simulink model "Simscape08"  (R2025b)
settings: Solver=ode23t  StartTime=0.0  StopTime=10  RelTol=1e-3
libraries: fl_lib x10, nesl_utility x4
settings Model: Creator=Nico6700  LastModifiedBy=Nico6700

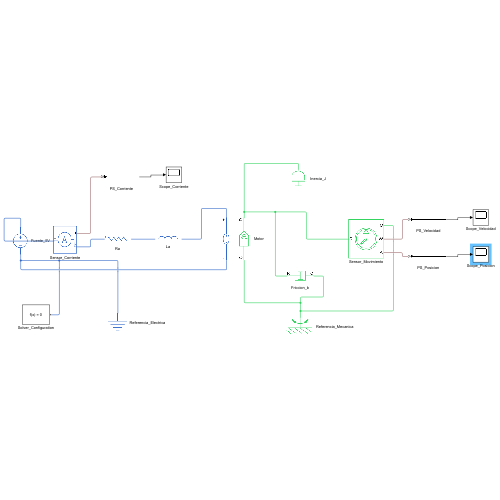
[thumbnail: Simulink's stored preview of the top-level diagram]
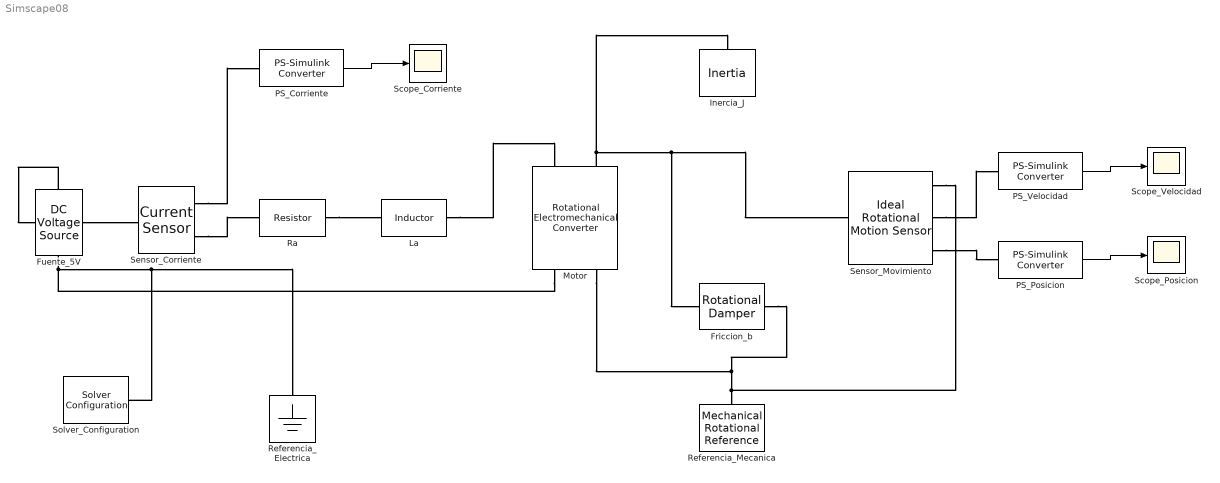
== system Simscape08 ==
  Friccion_b : fl_lib/Mechanical/Rotational Elements/Rotational Damper  D=0.0012 N*m*s/rad  w_specify=off  w_priority=None  w=0 rad/s  w_nominal_specify=off  w_nominal_value=1  w_nominal_unit=rad/s  t_specify=off  t_priority=None  t=0 N*m  t_nominal_specify=off  t_nominal_value=1  t_nominal_unit=N*m
  Fuente_5V : fl_lib/Electrical/Electrical Sources/DC Voltage Source  v0=5 V
  Inercia_J : fl_lib/Mechanical/Rotational Elements/Inertia  inertia=0.001 kg*m^2  num_ports=foundation.enum.numPorts2.one  w_specify=off  w_priority=High  w=0 rad/s  w_nominal_specify=off  w_nominal_value=1  w_nominal_unit=rad/s  t_specify=off  t_priority=None  t=0 N*m  t_nominal_specify=off  t_nominal_value=1  t_nominal_unit=N*m
  La : fl_lib/Electrical/Electrical Elements/Inductor  l=0.023 H  r=0 Ohm  g=1e-9 1/Ohm  i_specify=off  i_priority=None  i=0 A  i_nominal_specify=off  i_nominal_value=1  i_nominal_unit=A  v_specify=off  v_priority=None  v=0 V  v_nominal_specify=off  v_nominal_value=1  v_nominal_unit=V  i_L_specify=off  i_L_priority=High  i_L=0 A  i_L_nominal_specify=off  i_L_nominal_value=1  i_L_nominal_unit=A
  Motor : fl_lib/Electrical/Electrical Elements/Rotational Electromechanical Converter  K=0.01 V*s/rad  i_specify=off  i_priority=None  i=0 A  i_nominal_specify=off  i_nominal_value=1  i_nominal_unit=A  v_specify=off  v_priority=None  v=0 V  v_nominal_specify=off  v_nominal_value=1  v_nominal_unit=V  t_specify=off  t_priority=None  t=0 N*m  t_nominal_specify=off  t_nominal_value=1  t_nominal_unit=N*m  w_specify=off  w_priority=None  w=0 rad/s  w_nominal_specify=off  w_nominal_value=1  w_nominal_unit=rad/s
  PS_Corriente : nesl_utility/PS-Simulink Converter  PhysicalDomain=network_engine_domain  SubClassName=ps_output  LeftPortType=input  RightPortType=output  PseudoPeriodic=off  Frequencies=[]  VectorFormat=inherit  Unit=A  AffineConversion=off
  PS_Posicion : nesl_utility/PS-Simulink Converter  PhysicalDomain=network_engine_domain  SubClassName=ps_output  LeftPortType=input  RightPortType=output  PseudoPeriodic=off  Frequencies=[]  VectorFormat=inherit  Unit=rad  AffineConversion=off
  PS_Velocidad : nesl_utility/PS-Simulink Converter  PhysicalDomain=network_engine_domain  SubClassName=ps_output  LeftPortType=input  RightPortType=output  PseudoPeriodic=off  Frequencies=[]  VectorFormat=inherit  Unit=rad/s  AffineConversion=off
  Ra : fl_lib/Electrical/Electrical Elements/Resistor  R=2 Ohm  i_specify=off  i_priority=None  i=0 A  i_nominal_specify=off  i_nominal_value=1  i_nominal_unit=A  v_specify=off  v_priority=None  v=0 V  v_nominal_specify=off  v_nominal_value=1  v_nominal_unit=V
  Referencia_Electrica : fl_lib/Electrical/Electrical Elements/Electrical Reference
  Referencia_Mecanica : fl_lib/Mechanical/Rotational Elements/Mechanical Rotational Reference
  Scope_Corriente : Scope
      settings: ActiveDisplayYMinimum=-0.31140911926814757  ActiveDisplayYMaximum=2.8026821234133283
  Scope_Posicion : Scope
      settings: ActiveDisplayYMinimum=-22.972407166180481  ActiveDisplayYMaximum=206.75166449562437
  Scope_Velocidad : Scope
      settings: ActiveDisplayYMinimum=-2.499991028834232  ActiveDisplayYMaximum=22.49991925950809
  Sensor_Corriente : fl_lib/Electrical/Electrical Sensors/Current Sensor
  Sensor_Movimiento : fl_lib/Mechanical/Mechanical Sensors/Ideal Rotational Motion Sensor  reference=foundation.enum.MeasurementReference.difference  acceleration_port=false  velocity_port=true  position_port=true  wrap_angle=false  offset=0 rad
  Solver_Configuration : nesl_utility/Solver Configuration  PhysicalDomain=network_engine_domain  SubClassName=solver  LeftPortType=input  RightPortType=generic  Tones=[]  Harmonics=[]  SimulateNoise=off  Profile=off  UseLocalSampling=off  EnableSwitchedLinearOptims=on  FrequencyDomain=off  UseCCode=off  RelTol=0.001  AbsTol=0.001  MinStep=1e-09  ToWorkspace=off  RevertToSquareIcSolve=off  NumHomotopyIterations=100  PhasorMode=off  PhasorModeNumHarmonics=1  ConsistencySolver=NEWTON_XTOL_AFTER_FTOL  IndexReductionMethod=DerivativeReplacement  DoDC=off  ResidualTolerance=1e-09  ConsistencyTolSource=GLOBAL  ConsistencyAbsTol=0.001  ConsistencyRelTol=0.001  ConsistencyTolFactor=0.001  UseLocalSolver=off  LocalSolverChoice=NE_BACKWARD_EULER_ADVANCER  ResolveIndetEquations=on  FunctionEvalNumThread=1  LocalSolverSampleTime=0.001  DoFixedCost=off  MaxNonlinIter=3  MaxModeIter=2  ComputeImpulses=off  ImpulseIterations=2  LinearAlgebra=auto  LinearAlgebraNumThread=0  EquationFormulation=NE_TIME_EF  DelaysMemoryBudget=1024  AutomaticFiltering=on  FilteringTimeConstant=0.001  PartitionStorageMethod=AS_NEEDED  PartitionMemoryBudget=1024  PartitionMethod=ROBUST  MultibodyUseLocalSolver=off  MultibodyLocalSolverChoice=ODE1  MultibodyLocalSolverSampleTime=0.001
  wires:
  PS_Corriente/1 -> Scope_Corriente/1
  PS_Velocidad/1 -> Scope_Velocidad/1
  PS_Posicion/1 -> Scope_Posicion/1
  connections:
  Fuente_5V/LConn1 -- Sensor_Corriente/LConn1
  Sensor_Corriente/RConn2 -- Ra/LConn1
  Ra/RConn1 -- La/LConn1
  La/RConn1 -- Motor/LConn1
  Motor/RConn1 -- Solver_Configuration/RConn1 -- Referencia_Electrica/LConn1 -- Fuente_5V/RConn1
  Inercia_J/LConn1 -- Friccion_b/LConn1 -- Sensor_Movimiento/LConn1 -- Motor/LConn2
  Motor/RConn2 -- Friccion_b/RConn1 -- Referencia_Mecanica/LConn1 -- Sensor_Movimiento/RConn1
  Sensor_Corriente/RConn1 -- PS_Corriente/LConn1
  Sensor_Movimiento/RConn2 -- PS_Velocidad/LConn1
  Sensor_Movimiento/RConn3 -- PS_Posicion/LConn1
